simulink model "longitudinal_plant"  (R2026b)
settings: Solver=ode3  StopTime=10  FixedStep=P.sim.step
values from neighbouring files (symbols this model uses):
  P = initial_state(P, D, i0, sg_derivative(D.speed, D.t, 15))    [validate_longitudinal.m]
libraries: simulink x9, sl_discontinuities x2
settings Model: Creator=kikiw  LastModifiedBy=kikiw
settings DataIOCC: ExternalInput=u_ext  LoadExternalInput=on  SaveFormat=Array
settings OptimizationCC: BooleanDataType=off
settings DebuggingCC: AlgebraicLoopMsg=error

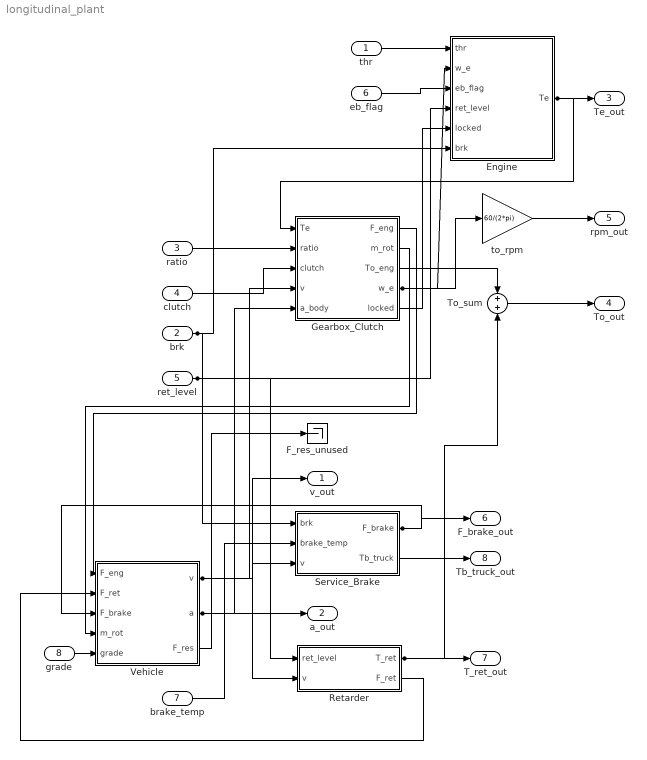
== system longitudinal_plant ==
  thr : Inport
  brk : Inport  Port=2
  ratio : Inport  Port=3
  clutch : Inport  Port=4
  ret_level : Inport  Port=5
  eb_flag : Inport  Port=6
  brake_temp : Inport  Port=7
  grade : Inport  Port=8
  Engine : Subsystem
  F_res_unused : Terminator
  Gearbox_Clutch : Subsystem
  Retarder : Subsystem
  Service_Brake : Subsystem
  To_sum : Sum
  Vehicle : Subsystem
  to_rpm : Gain  Gain=60/(2*pi)
  v_out : Outport
  a_out : Outport  Port=2
  Te_out : Outport  Port=3
  To_out : Outport  Port=4
  rpm_out : Outport  Port=5
  F_brake_out : Outport  Port=6
  T_ret_out : Outport  Port=7
  Tb_truck_out : Outport  Port=8
  wires:
  Vehicle/3(F_res) -> F_res_unused/1
  Vehicle/1(v) -> Gearbox_Clutch/4(v), Retarder/2(v), Service_Brake/3(v), v_out/1
  eb_flag/1 -> Engine/3(eb_flag)
  brake_temp/1 -> Service_Brake/2(brake_temp)
  grade/1 -> Vehicle/5(grade)
  ret_level/1 -> Engine/4(ret_level), Retarder/1(ret_level)
  thr/1 -> Engine/1(thr)
  ratio/1 -> Gearbox_Clutch/2(ratio)
  clutch/1 -> Gearbox_Clutch/3(clutch)
  brk/1 -> Engine/6(brk), Service_Brake/1(brk)
  Gearbox_Clutch/5(locked) -> Engine/5(locked)
  Vehicle/2(a) -> Gearbox_Clutch/5(a_body), a_out/1
  Gearbox_Clutch/1(F_eng) -> Vehicle/1(F_eng)
  Gearbox_Clutch/2(m_rot) -> Vehicle/4(m_rot)
  Gearbox_Clutch/3(To_eng) -> To_sum/1
  to_rpm/1 -> rpm_out/1
  Gearbox_Clutch/4(w_e) -> Engine/2(w_e), to_rpm/1
  Service_Brake/1(F_brake) -> Vehicle/3(F_brake), F_brake_out/1
  Service_Brake/2(Tb_truck) -> Tb_truck_out/1
  Retarder/1(T_ret) -> T_ret_out/1, To_sum/2
  Retarder/2(F_ret) -> Vehicle/2(F_ret)
  Engine/1(Te) -> Gearbox_Clutch/1(Te), Te_out/1
  To_sum/1 -> To_out/1

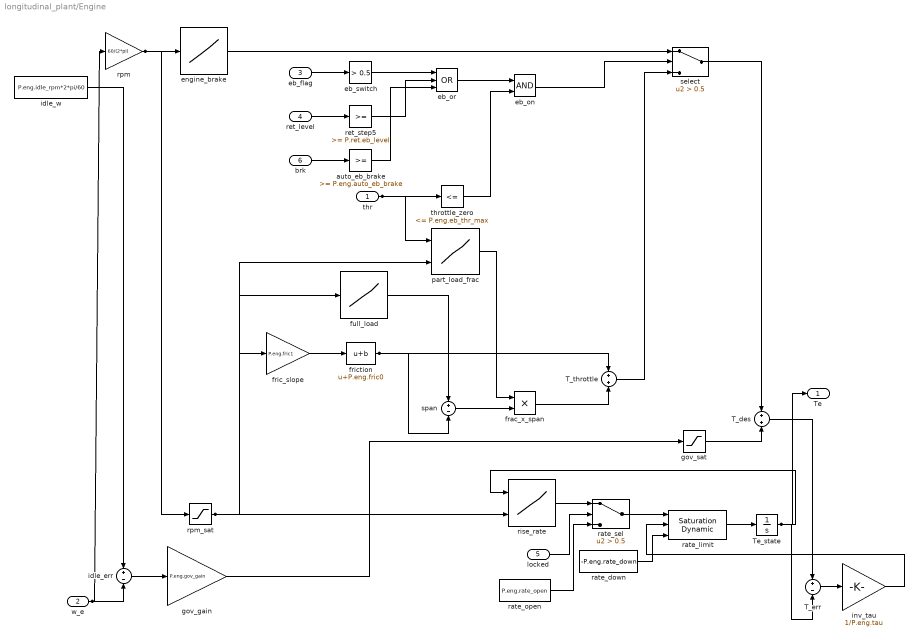
== system longitudinal_plant/Engine ==
  thr : Inport
  w_e : Inport  Port=2
  eb_flag : Inport  Port=3
  ret_level : Inport  Port=4
  locked : Inport  Port=5
  brk : Inport  Port=6
  T_des : Sum
  T_err : Sum  Inputs=+-
  T_throttle : Sum
  Te_state : Integrator  InitialCondition=P.init.Te0
  auto_eb_brake : simulink/Logic and Bit Operations/Compare To Constant  relop=>=  const=P.eng.auto_eb_brake  OutDataTypeStr=boolean
  eb_on : Logic  AllPortsSameDT=off  OutDataTypeStr=boolean
  eb_or : Logic  Operator=OR  Inputs=3  AllPortsSameDT=off  OutDataTypeStr=boolean
  eb_switch : simulink/Logic and Bit Operations/Compare To Constant  relop=>  const=0.5  OutDataTypeStr=boolean
  engine_brake : Lookup_n-D  NumberOfTableDimensions=1  BreakpointsForDimension1=P.eng.eb_rpm  Table=P.eng.eb_nm  ExtrapMethod=Clip  InternalRulePriority=Speed  RndMeth=Simplest
  frac_x_span : Product
  fric_slope : Gain  Gain=P.eng.fric1
  friction : Bias  Bias=P.eng.fric0  SaturateOnIntegerOverflow=off
  full_load : Lookup_n-D  NumberOfTableDimensions=1  BreakpointsForDimension1=P.eng.curve_rpm  Table=P.eng.T_max*P.eng.curve_frac  ExtrapMethod=Clip  InternalRulePriority=Speed  RndMeth=Simplest
  gov_gain : Gain  Gain=P.eng.gov_gain
  gov_sat : Saturate  UpperLimit=P.eng.T_max  LowerLimit=0
  idle_err : Sum  Inputs=+-
  idle_w : Constant  Value=P.eng.idle_rpm*2*pi/60
  inv_tau : Gain  Gain=1/P.eng.tau
  part_load_frac : Lookup_n-D  BreakpointsForDimension1=P.eng.thr_bp  BreakpointsForDimension2=P.eng.rpm_bp  Table=P.eng.frac_table  ExtrapMethod=Clip  InternalRulePriority=Speed  RndMeth=Simplest
      settings: InputPortMap=u0,u1
  rate_down : Constant  Value=-P.eng.rate_down
  rate_limit : sl_discontinuities/Saturation Dynamic  OutMin=[]  OutMax=[]  OutDataTypeStr=Inherit: Same as second input  OutDataType=fixdt(1, 16)  OutScaling=2^-10  DoSatur=off
      settings: LibrarySourceBlock=|
      | simulink/Discontinuities/Saturation
      | Dynamic
  rate_open : Constant  Value=P.eng.rate_open
  rate_sel : Switch  Criteria=u2 > Threshold  Threshold=0.5  SaturateOnIntegerOverflow=off  InputSameDT=off
  ret_step5 : simulink/Logic and Bit Operations/Compare To Constant  relop=>=  const=P.ret.eb_level  OutDataTypeStr=boolean
  rise_rate : Lookup_n-D  BreakpointsForDimension1=P.eng.rate_te_bp  BreakpointsForDimension2=P.eng.rate_rpm_bp  Table=P.eng.rate_up_table  ExtrapMethod=Clip  InternalRulePriority=Speed  RndMeth=Simplest
      settings: InputPortMap=u0,u1
  rpm : Gain  Gain=60/(2*pi)
  rpm_sat : Saturate  UpperLimit=P.eng.curve_rpm(end)  LowerLimit=P.eng.curve_rpm(1)
  select : Switch  Criteria=u2 > Threshold  Threshold=0.5  SaturateOnIntegerOverflow=off  InputSameDT=off
  span : Sum  Inputs=+-
  throttle_zero : simulink/Logic and Bit Operations/Compare To Constant  relop=<=  const=P.eng.eb_thr_max  OutDataTypeStr=boolean
  Te : Outport
  wires:
  idle_w/1 -> idle_err/1
  full_load/1 -> span/1
  rpm_sat/1 -> full_load/1, rise_rate/2, fric_slope/1, part_load_frac/2
  w_e/1 -> idle_err/2, rpm/1
  rpm/1 -> rpm_sat/1, engine_brake/1
  gov_gain/1 -> gov_sat/1
  T_des/1 -> T_err/1
  engine_brake/1 -> select/1
  T_throttle/1 -> select/3
  idle_err/1 -> gov_gain/1
  eb_flag/1 -> eb_switch/1
  ret_level/1 -> ret_step5/1
  brk/1 -> auto_eb_brake/1
  fric_slope/1 -> friction/1
  eb_switch/1 -> eb_or/1
  Te_state/1 -> T_err/2, rise_rate/1, Te/1
  ret_step5/1 -> eb_or/2
  auto_eb_brake/1 -> eb_or/3
  thr/1 -> part_load_frac/1, throttle_zero/1
  part_load_frac/1 -> frac_x_span/1
  friction/1 -> span/2, T_throttle/1
  eb_or/1 -> eb_on/1
  throttle_zero/1 -> eb_on/2
  frac_x_span/1 -> T_throttle/2
  span/1 -> frac_x_span/2
  eb_on/1 -> select/2
  rise_rate/1 -> rate_sel/1
  locked/1 -> rate_sel/2
  rate_open/1 -> rate_sel/3
  rate_sel/1 -> rate_limit/1
  T_err/1 -> inv_tau/1
  gov_sat/1 -> T_des/2
  rate_down/1 -> rate_limit/3
  select/1 -> T_des/1
  rate_limit/1 -> Te_state/1
  inv_tau/1 -> rate_limit/2

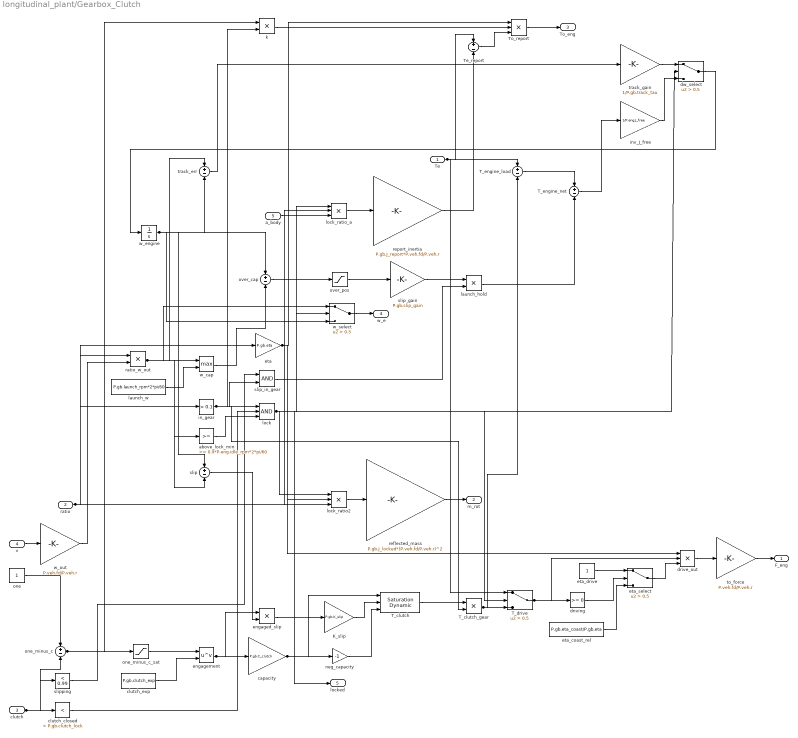
== system longitudinal_plant/Gearbox_Clutch ==
  Te : Inport
  ratio : Inport  Port=2
  clutch : Inport  Port=3
  v : Inport  Port=4
  a_body : Inport  Port=5
  K_slip : Gain  Gain=P.gb.K_slip
  T_clutch : sl_discontinuities/Saturation Dynamic  OutMin=[]  OutMax=[]  OutDataTypeStr=Inherit: Same as second input  OutDataType=fixdt(1, 16)  OutScaling=2^-10  DoSatur=off
      settings: LibrarySourceBlock=|
      | simulink/Discontinuities/Saturation
      | Dynamic
  T_clutch_gear : Product
  T_drive : Switch  Criteria=u2 > Threshold  Threshold=0.5  SaturateOnIntegerOverflow=off  InputSameDT=off
  T_engine_load : Sum  Inputs=+-
  T_engine_net : Sum  Inputs=+-
  Te_report : Sum  Inputs=+-
  To_report : Product  Inputs=3
  above_lock_min : simulink/Logic and Bit Operations/Compare To Constant  relop=>=  const=0.9*P.eng.idle_rpm*2*pi/60  OutDataTypeStr=boolean
  capacity : Gain  Gain=P.gb.C_clutch
  clutch_closed : simulink/Logic and Bit Operations/Compare To Constant  relop=<  const=P.gb.clutch_lock  OutDataTypeStr=boolean
  clutch_exp : Constant  Value=P.gb.clutch_exp
  drive_out : Product  Inputs=3
  driving : simulink/Logic and Bit Operations/Compare To Constant  relop=>=  const=0  OutDataTypeStr=boolean
  dw_select : Switch  Criteria=u2 > Threshold  Threshold=0.5  SaturateOnIntegerOverflow=off  InputSameDT=off
  engaged_slip : Product
  engagement : Math  Operator=pow
  eta : Gain  Gain=P.gb.eta
  eta_coast_rel : Constant  Value=P.gb.eta_coast/P.gb.eta
  eta_drive : Constant
  eta_select : Switch  Criteria=u2 > Threshold  Threshold=0.5  SaturateOnIntegerOverflow=off  InputSameDT=off
  in_gear : simulink/Logic and Bit Operations/Compare To Constant  relop=>  const=0.1  OutDataTypeStr=boolean
  inv_J_free : Gain  Gain=1/P.eng.J_free
  k : Product
  launch_hold : Product
  launch_w : Constant  Value=P.gb.launch_rpm*2*pi/60
  lock : Logic  Inputs=3  AllPortsSameDT=off  OutDataTypeStr=boolean
  lock_ratio2 : Product  Inputs=3
  lock_ratio_a : Product  Inputs=3
  neg_capacity : Gain  Gain=-1
  one : Constant
  one_minus_c : Sum  Inputs=+-
  one_minus_c_sat : Saturate  UpperLimit=1  LowerLimit=0
  over_cap : Sum  Inputs=+-
  over_pos : Saturate  UpperLimit=inf  LowerLimit=0
  ratio_w_out : Product
  reflected_mass : Gain  Gain=P.gb.J_locked*(P.veh.fd/P.veh.r)^2
  report_inertia : Gain  Gain=P.gb.J_report*P.veh.fd/P.veh.r
  slip : Sum  Inputs=+-
  slip_gain : Gain  Gain=P.gb.slip_gain
  slip_in_gear : Logic  AllPortsSameDT=off  OutDataTypeStr=boolean
  slipping : simulink/Logic and Bit Operations/Compare To Constant  relop=<  const=0.99  OutDataTypeStr=boolean
  to_force : Gain  Gain=P.veh.fd/P.veh.r
  track_err : Sum  Inputs=+-
  track_gain : Gain  Gain=1/P.gb.track_tau
  w_cap : MinMax  Function=max  Inputs=2
  w_engine : Integrator  InitialCondition=P.init.we0  LimitOutput=on  UpperSaturationLimit=P.eng.max_rpm*2*pi/60  LowerSaturationLimit=0
  w_out : Gain  Gain=P.veh.fd/P.veh.r
  w_select : Switch  Criteria=u2 > Threshold  Threshold=0.5  SaturateOnIntegerOverflow=off  InputSameDT=off
  F_eng : Outport
  m_rot : Outport  Port=2
  To_eng : Outport  Port=3
  w_e : Outport  Port=4
  locked : Outport  Port=5
  wires:
  v/1 -> w_out/1
  slip_in_gear/1 -> launch_hold/2
  above_lock_min/1 -> lock/3
  clutch_closed/1 -> lock/2
  over_pos/1 -> slip_gain/1
  w_cap/1 -> over_cap/2
  one/1 -> one_minus_c/1
  ratio/1 -> in_gear/1, eta/1, lock_ratio2/3, ratio_w_out/1, lock_ratio_a/2
  slipping/1 -> slip_in_gear/1
  over_cap/1 -> over_pos/1
  clutch/1 -> one_minus_c/2, clutch_closed/1, slipping/1
  inv_J_free/1 -> dw_select/3
  w_out/1 -> ratio_w_out/2
  one_minus_c/1 -> k/1, one_minus_c_sat/1
  w_engine/1 -> w_select/3, over_cap/1, slip/1, track_err/2
  K_slip/1 -> T_clutch/2
  ratio_w_out/1 -> track_err/1, w_select/1, slip/2, above_lock_min/1, w_cap/1
  launch_w/1 -> w_cap/2
  one_minus_c_sat/1 -> engagement/1
  clutch_exp/1 -> engagement/2
  track_err/1 -> track_gain/1
  in_gear/1 -> lock/1, k/2, T_clutch_gear/2, slip_in_gear/2
  slip/1 -> engaged_slip/2
  engagement/1 -> engaged_slip/1, capacity/1
  k/1 -> To_report/2
  a_body/1 -> lock_ratio_a/3
  eta/1 -> drive_out/1, To_report/1, lock_ratio2/2
  reflected_mass/1 -> m_rot/1
  lock/1 -> T_drive/2, dw_select/2, lock_ratio_a/1, w_select/2, lock_ratio2/1, locked/1
  track_gain/1 -> dw_select/1
  engaged_slip/1 -> K_slip/1
  capacity/1 -> T_clutch/1, neg_capacity/1
  lock_ratio2/1 -> reflected_mass/1
  lock_ratio_a/1 -> report_inertia/1
  dw_select/1 -> w_engine/1
  w_select/1 -> w_e/1
  neg_capacity/1 -> T_clutch/3
  Te/1 -> T_drive/1, Te_report/1, T_engine_load/1
  report_inertia/1 -> Te_report/2
  slip_gain/1 -> launch_hold/1
  T_clutch/1 -> T_clutch_gear/1
  Te_report/1 -> To_report/3
  T_clutch_gear/1 -> T_engine_load/2, T_drive/3
  launch_hold/1 -> T_engine_net/2
  eta_select/1 -> drive_out/3
  To_report/1 -> To_eng/1
  T_drive/1 -> drive_out/2, driving/1
  T_engine_load/1 -> T_engine_net/1
  T_engine_net/1 -> inv_J_free/1
  eta_drive/1 -> eta_select/1
  driving/1 -> eta_select/2
  eta_coast_rel/1 -> eta_select/3
  drive_out/1 -> to_force/1
  to_force/1 -> F_eng/1

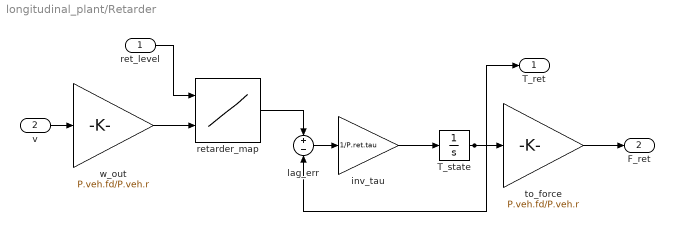
== system longitudinal_plant/Retarder ==
  ret_level : Inport
  v : Inport  Port=2
  T_state : Integrator  InitialCondition=P.init.ret0
  inv_tau : Gain  Gain=1/P.ret.tau
  lag_err : Sum  Inputs=+-
  retarder_map : Lookup_n-D  BreakpointsForDimension1=P.ret.level_bp  BreakpointsForDimension2=P.ret.w_bp  Table=P.ret.table  ExtrapMethod=Clip  InternalRulePriority=Speed  RndMeth=Simplest
      settings: InputPortMap=u0,u1
  to_force : Gain  Gain=P.veh.fd/P.veh.r
  w_out : Gain  Gain=P.veh.fd/P.veh.r
  T_ret : Outport
  F_ret : Outport  Port=2
  wires:
  v/1 -> w_out/1
  ret_level/1 -> retarder_map/1
  T_state/1 -> lag_err/2, T_ret/1, to_force/1
  retarder_map/1 -> lag_err/1
  w_out/1 -> retarder_map/2
  lag_err/1 -> inv_tau/1
  to_force/1 -> F_ret/1
  inv_tau/1 -> T_state/1

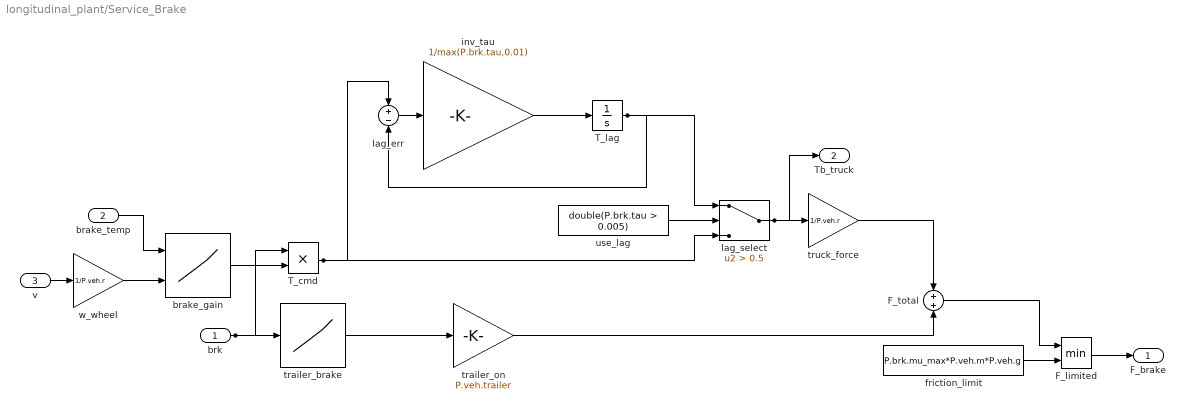
== system longitudinal_plant/Service_Brake ==
  brk : Inport
  brake_temp : Inport  Port=2
  v : Inport  Port=3
  F_limited : MinMax  Inputs=2
  F_total : Sum
  T_cmd : Product
  T_lag : Integrator
  brake_gain : Lookup_n-D  BreakpointsForDimension1=P.brk.temp_bp  BreakpointsForDimension2=P.brk.w_bp  Table=P.brk.gain_table  ExtrapMethod=Clip  InternalRulePriority=Speed  RndMeth=Simplest
      settings: InputPortMap=u0,u1
  friction_limit : Constant  Value=P.brk.mu_max*P.veh.m*P.veh.g
  inv_tau : Gain  Gain=1/max(P.brk.tau,0.01)
  lag_err : Sum  Inputs=+-
  lag_select : Switch  Criteria=u2 > Threshold  Threshold=0.5  SaturateOnIntegerOverflow=off  InputSameDT=off
  trailer_brake : Lookup_n-D  NumberOfTableDimensions=1  BreakpointsForDimension1=P.brk.trailer_bp  Table=P.brk.trailer_force  ExtrapMethod=Clip  InternalRulePriority=Speed  RndMeth=Simplest
  trailer_on : Gain  Gain=P.veh.trailer
  truck_force : Gain  Gain=1/P.veh.r
  use_lag : Constant  Value=double(P.brk.tau > 0.005)
  w_wheel : Gain  Gain=1/P.veh.r
  F_brake : Outport
  Tb_truck : Outport  Port=2
  wires:
  truck_force/1 -> F_total/1
  lag_err/1 -> inv_tau/1
  w_wheel/1 -> brake_gain/2
  T_cmd/1 -> lag_err/1, lag_select/3
  brake_gain/1 -> T_cmd/2
  v/1 -> w_wheel/1
  trailer_brake/1 -> trailer_on/1
  F_limited/1 -> F_brake/1
  brake_temp/1 -> brake_gain/1
  friction_limit/1 -> F_limited/2
  brk/1 -> T_cmd/1, trailer_brake/1
  inv_tau/1 -> T_lag/1
  T_lag/1 -> lag_err/2, lag_select/1
  trailer_on/1 -> F_total/2
  use_lag/1 -> lag_select/2
  lag_select/1 -> truck_force/1, Tb_truck/1
  F_total/1 -> F_limited/1

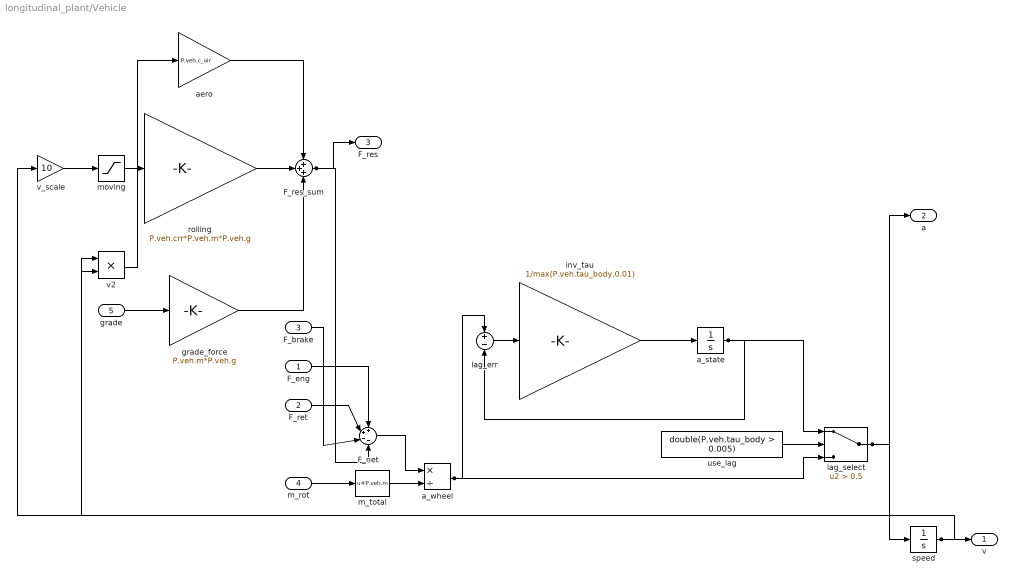
== system longitudinal_plant/Vehicle ==
  F_eng : Inport
  F_ret : Inport  Port=2
  F_brake : Inport  Port=3
  m_rot : Inport  Port=4
  grade : Inport  Port=5
  F_net : Sum  Inputs=++--
  F_res_sum : Sum  Inputs=+++
  a_state : Integrator  InitialCondition=P.init.a0
  a_wheel : Product  Inputs=*/
  aero : Gain  Gain=P.veh.c_air
  grade_force : Gain  Gain=P.veh.m*P.veh.g
  inv_tau : Gain  Gain=1/max(P.veh.tau_body,0.01)
  lag_err : Sum  Inputs=+-
  lag_select : Switch  Criteria=u2 > Threshold  Threshold=0.5  SaturateOnIntegerOverflow=off  InputSameDT=off
  m_total : Bias  Bias=P.veh.m  SaturateOnIntegerOverflow=off
  moving : Saturate  UpperLimit=1  LowerLimit=0
  rolling : Gain  Gain=P.veh.crr*P.veh.m*P.veh.g
  speed : Integrator  InitialCondition=P.init.v0  LimitOutput=on  LowerSaturationLimit=0
  use_lag : Constant  Value=double(P.veh.tau_body > 0.005)
  v2 : Product
  v_scale : Gain  Gain=10
  v : Outport
  a : Outport  Port=2
  F_res : Outport  Port=3
  wires:
  v_scale/1 -> moving/1
  aero/1 -> F_res_sum/1
  moving/1 -> rolling/1
  grade/1 -> grade_force/1
  v2/1 -> aero/1
  rolling/1 -> F_res_sum/2
  F_res_sum/1 -> F_net/4, F_res/1
  grade_force/1 -> F_res_sum/3
  F_brake/1 -> F_net/3
  F_eng/1 -> F_net/1
  F_ret/1 -> F_net/2
  m_rot/1 -> m_total/1
  inv_tau/1 -> a_state/1
  F_net/1 -> a_wheel/1
  use_lag/1 -> lag_select/2
  m_total/1 -> a_wheel/2
  a_wheel/1 -> lag_err/1, lag_select/3
  speed/1 -> v2/1, v_scale/1, v2/2, v/1
  lag_err/1 -> inv_tau/1
  a_state/1 -> lag_err/2, lag_select/1
  lag_select/1 -> speed/1, a/1
